simulink model "MMC_phase_centralized_HAAS_20260927"  (R2024b)
settings: Solver=FixedStepDiscrete  StartTime=t_init_sim  StopTime=sim_time  FixedStep=Ts  RelTol=1e-3
values from neighbouring files (symbols this model uses):
  a = 1    [script_MMC_phase_hackathon_NLM_centralized_HAAS_20260927.m]
  C1low1_active = 1    [script_MMC_phase_hackathon_NLM_centralized_HAAS_20260927.m]
  C2low1_active = 1    [script_MMC_phase_hackathon_NLM_centralized_HAAS_20260927.m]
  C_bus = 4400e-6    (= 0.0044)    [script_MMC_phase_hackathon_NLM_centralized_HAAS_20260927.m]
  C_M_extra = C_m-twist_high_side_C    [script_MMC_phase_hackathon_NLM_centralized_HAAS_20260927.m]
  duty_cycle = 1.0    (= 1)    [script_MMC_phase_hackathon_NLM_centralized_HAAS_20260927.m]
  f0 = 50    [script_MMC_phase_hackathon_NLM_centralized_HAAS_20260927.m]
  feeder_current_lower_rate_limit = -10    [script_MMC_phase_hackathon_NLM_centralized_HAAS_20260927.m]    (also in twist_parameters.m = -500)
  feeder_current_tab = [0.328 0.217 0.162 0.132 0.109 0.094 0.083 0.075 0.068 0.062 0.058 0.054 ... (42 elements, 14x3)]    [feeder_current.mat]
  feeder_current_upper_rate_limit = 0.386/(20e-3)    (= 19.3)    [twist_parameters.m]
  is6VExternallySupplied = true    [script_MMC_phase_hackathon_NLM_centralized_HAAS_20260927.m]
  isFeederJumperOpen = true    [script_MMC_phase_hackathon_NLM_centralized_HAAS_20260927.m]
  L_arm = 30e-3    (= 0.03)    [script_MMC_phase_hackathon_NLM_centralized_HAAS_20260927.m]
  m = 1    [script_MMC_phase_hackathon_NLM_centralized_HAAS_20260927.m]
  N = 5    [script_MMC_phase_hackathon_NLM_centralized_HAAS_20260927.m]
  power_losses = false    [script_MMC_phase_hackathon_NLM_centralized_HAAS_20260927.m]
  R = 15    [script_MMC_phase_hackathon_NLM_centralized_HAAS_20260927.m]
  R_arm = 0.2    [script_MMC_phase_hackathon_NLM_centralized_HAAS_20260927.m]
  source_V = 0    [script_MMC_phase_hackathon_NLM_centralized_HAAS_20260927.m]
  Tcom_sample = round(Tcom / Ts)    [script_MMC_phase_hackathon_NLM_centralized_HAAS_20260927.m]
  time_charge = 0.1    [script_MMC_phase_hackathon_NLM_centralized_HAAS_20260927.m]
  time_decharge = 1.5    [script_MMC_phase_hackathon_NLM_centralized_HAAS_20260927.m]
  Ts = 1e-6    (= 1e-06)    [script_MMC_phase_hackathon_NLM_centralized_HAAS_20260927.m]
  twist_data_acquisition_delay = 50e-9    (= 5e-08)    [script_MMC_phase_hackathon_NLM_centralized_HAAS_20260927.m]    (also in twist_parameters.m)
  twist_data_sampling_period = 1/twist_freq_data_sampling    (= 5e-05)    [script_MMC_phase_hackathon_NLM_centralized_HAAS_20260927.m]    (also in twist_parameters.m)
  twist_dead_time = 200e-9    (= 2e-07)    [twist_parameters.m]
  twist_freq_switching = 200e3    (= 200000)    [twist_parameters.m]
  twist_high_side_adc_R = 1/(1/2e6 + 1/2e6 + 1/(330e3+5.6e3))    (= 251272.836178)    [twist_parameters.m]
  twist_high_side_C = 33e-6*4 + 4.7e-6*12    (= 0.0001884)    [twist_parameters.m]
  twist_high_side_feeder_R = 47e3+4.7e3    (= 51700)    [twist_parameters.m]
  twist_high_side_rC = 0.1    [twist_parameters.m]
  twist_low_side_adc_R = 150e3+470    (= 150470)    [twist_parameters.m]
  twist_low_side_C_ceramic = 3*4.7e-6    (= 1.41e-05)    [twist_parameters.m]
  twist_low_side_C_electrolytic = 47e-6    (= 4.7e-05)    [twist_parameters.m]
  twist_low_side_L = 33e-6    (= 3.3e-05)    [twist_parameters.m]
  twist_low_side_rC = 700e-3    (= 0.7)    [twist_parameters.m]
  twist_low_side_rL = 20e-3    (= 0.02)    [twist_parameters.m]
  twist_R_VCC = (tau_VCC/twist_high_side_C  - twist_high_side_rC)/(1-(tau_VCC/twist_high_side_C - twist_high_side_rC)/R_parallel)    (= 1110.74997822)    [twist_parameters.m]
  VDC = 48    [script_MMC_phase_hackathon_NLM_centralized_HAAS_20260927.m]
undefined symbols (not defined in the file or in its folder): C_SM, feeder_current, gcbh, sps_rtmsupport, twist_low_side_lC
libraries: spsSeriesRLCBranchLib x135, spsTriangleGeneratorLib x60, spsMosfetLib x60, spsCurrentMeasurementLib x43, spsVoltageMeasurementLib x35, spsControlledCurrentSourceLib x30, spsDiodeLib x22, spsIdealSwitchLib x20, spsControlledVoltageSourceLib x1, spsGroundLib x1, spspowerguiLib x1
(part 10 of 22)

== system MMC_phase_centralized_HAAS_20260927/ /Subsystem/Subsystem/Hardware M2/Measurement block/i2Low acquisition ==
  In1 : Inport
  In2 : Inport  Port=2
  If : If  IfExpression=u1 > 0.99  ShowElse=off
  If Action Subsystem : Subsystem  TreatAsAtomicUnit=on
  Scope : Scope  NumInputPorts=3
  i2Meas : Outport
  wires:
  If Action Subsystem/1(Out1) -> Scope/1, i2Meas/1  "Data_Carry"
  In1/1 -> Scope/2, If Action Subsystem/1(In1)  "Data"
  If/1 -> If Action Subsystem/Action
  In2/1 -> If/1, Scope/3  "Carry"

== system MMC_phase_centralized_HAAS_20260927/ /Subsystem/Subsystem/Hardware M2/Measurement block/iHigh acquisition ==
  In1 : Inport
  In2 : Inport  Port=2
  If : If  IfExpression=u1 > 0.99  ShowElse=off
  If Action Subsystem : Subsystem  TreatAsAtomicUnit=on
  Scope : Scope  NumInputPorts=3
  iHMeas : Outport
  wires:
  If Action Subsystem/1(Out1) -> Scope/1, iHMeas/1  "Data_Carry"
  In1/1 -> Scope/2, If Action Subsystem/1(In1)  "Data"
  If/1 -> If Action Subsystem/Action
  In2/1 -> If/1, Scope/3  "Carry"

== system MMC_phase_centralized_HAAS_20260927/ /Subsystem/Subsystem/Hardware M2/Measurement block/v1Low acquisition ==
  In1 : Inport
  In2 : Inport  Port=2
  If : If  IfExpression=u1 > 0.99  ShowElse=off
  If Action Subsystem : Subsystem  TreatAsAtomicUnit=on
  Scope : Scope  NumInputPorts=3
  v1Meas : Outport
  wires:
  If Action Subsystem/1(Out1) -> Scope/1, v1Meas/1  "Data_Carry"
  In1/1 -> Scope/2, If Action Subsystem/1(In1)  "Data"
  If/1 -> If Action Subsystem/Action
  In2/1 -> If/1, Scope/3  "Carry"

== system MMC_phase_centralized_HAAS_20260927/ /Subsystem/Subsystem/Hardware M2/Measurement block/v2Low acquisition ==
  In1 : Inport
  In2 : Inport  Port=2
  If : If  IfExpression=u1 > 0.99  ShowElse=off
  If Action Subsystem : Subsystem  TreatAsAtomicUnit=on
  Scope : Scope  NumInputPorts=3
  v2Meas : Outport
  wires:
  If Action Subsystem/1(Out1) -> Scope/1, v2Meas/1  "Data_Carry"
  In1/1 -> Scope/2, If Action Subsystem/1(In1)  "Data"
  If/1 -> If Action Subsystem/Action
  In2/1 -> If/1, Scope/3  "Carry"

== system MMC_phase_centralized_HAAS_20260927/ /Subsystem/Subsystem/Hardware M2/Measurement block/vHigh acquisition ==
  In1 : Inport
  In2 : Inport  Port=2
  If : If  IfExpression=u1 > 0.99  ShowElse=off
  If Action Subsystem : Subsystem  TreatAsAtomicUnit=on
  Scope : Scope  NumInputPorts=3
  vHMeas : Outport
  wires:
  If Action Subsystem/1(Out1) -> Scope/1, vHMeas/1  "Data_Carry"
  In1/1 -> Scope/2, If Action Subsystem/1(In1)  "Data"
  If/1 -> If Action Subsystem/Action
  In2/1 -> If/1, Scope/3  "Carry"

== system MMC_phase_centralized_HAAS_20260927/ /Subsystem/Subsystem/Hardware M3/HRTimA_1/PWM Generator (2-Level) ==
  Uref : Inport  PortDimensions=sps.UrefInport_PortDimensions  SampleTime=Ts
  Bus Creator : BusCreator  Inputs=2
  Constant10 : Constant  Value=MinMax
  Cr_MinMax : Subsystem
  Data Type Conversion : DataTypeConversion  OutDataTypeStr=double  SaturateOnIntegerOverflow=off  RndMeth=Floor
  Logical Operator4 : Logic  Operator=NOT
  Modulator type : Subsystem  BlockChoice=One_Three_PhaseBridge  Variant=on  VariantControlMode=label  LabelModeActiveChoice=OneThreePhaseBridge
  Mux3 : Mux  Inputs=2
  Reference signal : Subsystem  BlockChoice=InternalUref  Variant=on  VariantControlMode=label  LabelModeActiveChoice=External
  Sampling : Subsystem  BlockChoice=Unsync_NaturalSampling  Variant=on  VariantControlMode=label  LabelModeActiveChoice=UnsyncSymmetrical
  Selector_Pout : Selector  InputPortWidth=sps.SelectorPout_PortSize  IndexOptions=Index vector (dialog)  Indices=sps.SelectorPout_Index  OutputSizes=1
  m : Terminator
  wt : Ground
  P : Outport  SampleTime=Ts  VectorParamsAs1DForOutWhenUnconnected=off
  Carry : Outport  Port=2  SampleTime=Ts  VectorParamsAs1DForOutWhenUnconnected=off
  wires:
  wt/1 -> Sampling/1(wt)
  Reference signal/1(Uref_In) -> Sampling/2(Uref)
  Modulator type/1(P) -> Logical Operator4/1, Mux3/1
  Constant10/1 -> Cr_MinMax/1(MinMax)
  Uref/1 -> Reference signal/1(Uref)
  Data Type Conversion/1 -> P/1
  Logical Operator4/1 -> Mux3/2
  Mux3/1 -> Selector_Pout/1
  Selector_Pout/1 -> Data Type Conversion/1
  Cr_MinMax/1(Cr*) -> Carry/1, Bus Creator/1, Modulator type/1(Cr)  "carrier"
  Sampling/1(Cr) -> Cr_MinMax/2(Cr)
  Sampling/2(Uref*) -> Bus Creator/2, Modulator type/2(Uref)  "Uref"
  Bus Creator/1 -> m/1

== system MMC_phase_centralized_HAAS_20260927/ /Subsystem/Subsystem/Hardware M3/HRTimA_2/PWM Generator (2-Level) ==
  Uref : Inport  PortDimensions=sps.UrefInport_PortDimensions  SampleTime=Ts
  Bus Creator : BusCreator  Inputs=2
  Constant10 : Constant  Value=MinMax
  Cr_MinMax : Subsystem
  Data Type Conversion : DataTypeConversion  OutDataTypeStr=double  SaturateOnIntegerOverflow=off  RndMeth=Floor
  Logical Operator4 : Logic  Operator=NOT
  Modulator type : Subsystem  BlockChoice=One_Three_PhaseBridge  Variant=on  VariantControlMode=label  LabelModeActiveChoice=OneThreePhaseBridge
  Mux3 : Mux  Inputs=2
  Reference signal : Subsystem  BlockChoice=InternalUref  Variant=on  VariantControlMode=label  LabelModeActiveChoice=External
  Sampling : Subsystem  BlockChoice=Unsync_NaturalSampling  Variant=on  VariantControlMode=label  LabelModeActiveChoice=UnsyncSymmetrical
  Selector_Pout : Selector  InputPortWidth=sps.SelectorPout_PortSize  IndexOptions=Index vector (dialog)  Indices=sps.SelectorPout_Index  OutputSizes=1
  m : Terminator
  wt : Ground
  P : Outport  SampleTime=Ts  VectorParamsAs1DForOutWhenUnconnected=off
  Carry : Outport  Port=2  SampleTime=Ts  VectorParamsAs1DForOutWhenUnconnected=off
  wires:
  wt/1 -> Sampling/1(wt)
  Reference signal/1(Uref_In) -> Sampling/2(Uref)
  Modulator type/1(P) -> Logical Operator4/1, Mux3/1
  Constant10/1 -> Cr_MinMax/1(MinMax)
  Uref/1 -> Reference signal/1(Uref)
  Data Type Conversion/1 -> P/1
  Logical Operator4/1 -> Mux3/2
  Mux3/1 -> Selector_Pout/1
  Selector_Pout/1 -> Data Type Conversion/1
  Cr_MinMax/1(Cr*) -> Carry/1, Bus Creator/1, Modulator type/1(Cr)  "carrier"
  Sampling/1(Cr) -> Cr_MinMax/2(Cr)
  Sampling/2(Uref*) -> Bus Creator/2, Modulator type/2(Uref)  "Uref"
  Bus Creator/1 -> m/1

== system MMC_phase_centralized_HAAS_20260927/ /Subsystem/Subsystem/Hardware M3/Measurement block/i1Low acquisition ==
  In1 : Inport
  In2 : Inport  Port=2
  If : If  IfExpression=u1 > 0.99  ShowElse=off
  If Action Subsystem : Subsystem  TreatAsAtomicUnit=on
  Scope : Scope  NumInputPorts=3
  i1Meas : Outport
  wires:
  If Action Subsystem/1(Out1) -> Scope/1, i1Meas/1  "Data_Carry"
  In1/1 -> Scope/2, If Action Subsystem/1(In1)  "Data"
  If/1 -> If Action Subsystem/Action
  In2/1 -> If/1, Scope/3  "Carry"

== system MMC_phase_centralized_HAAS_20260927/ /Subsystem/Subsystem/Hardware M3/Measurement block/i2Low acquisition ==
  In1 : Inport
  In2 : Inport  Port=2
  If : If  IfExpression=u1 > 0.99  ShowElse=off
  If Action Subsystem : Subsystem  TreatAsAtomicUnit=on
  Scope : Scope  NumInputPorts=3
  i2Meas : Outport
  wires:
  If Action Subsystem/1(Out1) -> Scope/1, i2Meas/1  "Data_Carry"
  In1/1 -> Scope/2, If Action Subsystem/1(In1)  "Data"
  If/1 -> If Action Subsystem/Action
  In2/1 -> If/1, Scope/3  "Carry"

== system MMC_phase_centralized_HAAS_20260927/ /Subsystem/Subsystem/Hardware M3/Measurement block/iHigh acquisition ==
  In1 : Inport
  In2 : Inport  Port=2
  If : If  IfExpression=u1 > 0.99  ShowElse=off
  If Action Subsystem : Subsystem  TreatAsAtomicUnit=on
  Scope : Scope  NumInputPorts=3
  iHMeas : Outport
  wires:
  If Action Subsystem/1(Out1) -> Scope/1, iHMeas/1  "Data_Carry"
  In1/1 -> Scope/2, If Action Subsystem/1(In1)  "Data"
  If/1 -> If Action Subsystem/Action
  In2/1 -> If/1, Scope/3  "Carry"

== system MMC_phase_centralized_HAAS_20260927/ /Subsystem/Subsystem/Hardware M3/Measurement block/v1Low acquisition ==
  In1 : Inport
  In2 : Inport  Port=2
  If : If  IfExpression=u1 > 0.99  ShowElse=off
  If Action Subsystem : Subsystem  TreatAsAtomicUnit=on
  Scope : Scope  NumInputPorts=3
  v1Meas : Outport
  wires:
  If Action Subsystem/1(Out1) -> Scope/1, v1Meas/1  "Data_Carry"
  In1/1 -> Scope/2, If Action Subsystem/1(In1)  "Data"
  If/1 -> If Action Subsystem/Action
  In2/1 -> If/1, Scope/3  "Carry"

== system MMC_phase_centralized_HAAS_20260927/ /Subsystem/Subsystem/Hardware M3/Measurement block/v2Low acquisition ==
  In1 : Inport
  In2 : Inport  Port=2
  If : If  IfExpression=u1 > 0.99  ShowElse=off
  If Action Subsystem : Subsystem  TreatAsAtomicUnit=on
  Scope : Scope  NumInputPorts=3
  v2Meas : Outport
  wires:
  If Action Subsystem/1(Out1) -> Scope/1, v2Meas/1  "Data_Carry"
  In1/1 -> Scope/2, If Action Subsystem/1(In1)  "Data"
  If/1 -> If Action Subsystem/Action
  In2/1 -> If/1, Scope/3  "Carry"

== system MMC_phase_centralized_HAAS_20260927/ /Subsystem/Subsystem/Hardware M3/Measurement block/vHigh acquisition ==
  In1 : Inport
  In2 : Inport  Port=2
  If : If  IfExpression=u1 > 0.99  ShowElse=off
  If Action Subsystem : Subsystem  TreatAsAtomicUnit=on
  Scope : Scope  NumInputPorts=3
  vHMeas : Outport
  wires:
  If Action Subsystem/1(Out1) -> Scope/1, vHMeas/1  "Data_Carry"
  In1/1 -> Scope/2, If Action Subsystem/1(In1)  "Data"
  If/1 -> If Action Subsystem/Action
  In2/1 -> If/1, Scope/3  "Carry"

== system MMC_phase_centralized_HAAS_20260927/ /Subsystem/Subsystem/Hardware M4/HRTimA_1/PWM Generator (2-Level) ==
  Uref : Inport  PortDimensions=sps.UrefInport_PortDimensions  SampleTime=Ts
  Bus Creator : BusCreator  Inputs=2
  Constant10 : Constant  Value=MinMax
  Cr_MinMax : Subsystem
  Data Type Conversion : DataTypeConversion  OutDataTypeStr=double  SaturateOnIntegerOverflow=off  RndMeth=Floor
  Logical Operator4 : Logic  Operator=NOT
  Modulator type : Subsystem  BlockChoice=One_Three_PhaseBridge  Variant=on  VariantControlMode=label  LabelModeActiveChoice=OneThreePhaseBridge
  Mux3 : Mux  Inputs=2
  Reference signal : Subsystem  BlockChoice=InternalUref  Variant=on  VariantControlMode=label  LabelModeActiveChoice=External
  Sampling : Subsystem  BlockChoice=Unsync_NaturalSampling  Variant=on  VariantControlMode=label  LabelModeActiveChoice=UnsyncSymmetrical
  Selector_Pout : Selector  InputPortWidth=sps.SelectorPout_PortSize  IndexOptions=Index vector (dialog)  Indices=sps.SelectorPout_Index  OutputSizes=1
  m : Terminator
  wt : Ground
  P : Outport  SampleTime=Ts  VectorParamsAs1DForOutWhenUnconnected=off
  Carry : Outport  Port=2  SampleTime=Ts  VectorParamsAs1DForOutWhenUnconnected=off
  wires:
  wt/1 -> Sampling/1(wt)
  Reference signal/1(Uref_In) -> Sampling/2(Uref)
  Modulator type/1(P) -> Logical Operator4/1, Mux3/1
  Constant10/1 -> Cr_MinMax/1(MinMax)
  Uref/1 -> Reference signal/1(Uref)
  Data Type Conversion/1 -> P/1
  Logical Operator4/1 -> Mux3/2
  Mux3/1 -> Selector_Pout/1
  Selector_Pout/1 -> Data Type Conversion/1
  Cr_MinMax/1(Cr*) -> Carry/1, Bus Creator/1, Modulator type/1(Cr)  "carrier"
  Sampling/1(Cr) -> Cr_MinMax/2(Cr)
  Sampling/2(Uref*) -> Bus Creator/2, Modulator type/2(Uref)  "Uref"
  Bus Creator/1 -> m/1

== system MMC_phase_centralized_HAAS_20260927/ /Subsystem/Subsystem/Hardware M4/HRTimA_2/PWM Generator (2-Level) ==
  Uref : Inport  PortDimensions=sps.UrefInport_PortDimensions  SampleTime=Ts
  Bus Creator : BusCreator  Inputs=2
  Constant10 : Constant  Value=MinMax
  Cr_MinMax : Subsystem
  Data Type Conversion : DataTypeConversion  OutDataTypeStr=double  SaturateOnIntegerOverflow=off  RndMeth=Floor
  Logical Operator4 : Logic  Operator=NOT
  Modulator type : Subsystem  BlockChoice=One_Three_PhaseBridge  Variant=on  VariantControlMode=label  LabelModeActiveChoice=OneThreePhaseBridge
  Mux3 : Mux  Inputs=2
  Reference signal : Subsystem  BlockChoice=InternalUref  Variant=on  VariantControlMode=label  LabelModeActiveChoice=External
  Sampling : Subsystem  BlockChoice=Unsync_NaturalSampling  Variant=on  VariantControlMode=label  LabelModeActiveChoice=UnsyncSymmetrical
  Selector_Pout : Selector  InputPortWidth=sps.SelectorPout_PortSize  IndexOptions=Index vector (dialog)  Indices=sps.SelectorPout_Index  OutputSizes=1
  m : Terminator
  wt : Ground
  P : Outport  SampleTime=Ts  VectorParamsAs1DForOutWhenUnconnected=off
  Carry : Outport  Port=2  SampleTime=Ts  VectorParamsAs1DForOutWhenUnconnected=off
  wires:
  wt/1 -> Sampling/1(wt)
  Reference signal/1(Uref_In) -> Sampling/2(Uref)
  Modulator type/1(P) -> Logical Operator4/1, Mux3/1
  Constant10/1 -> Cr_MinMax/1(MinMax)
  Uref/1 -> Reference signal/1(Uref)
  Data Type Conversion/1 -> P/1
  Logical Operator4/1 -> Mux3/2
  Mux3/1 -> Selector_Pout/1
  Selector_Pout/1 -> Data Type Conversion/1
  Cr_MinMax/1(Cr*) -> Carry/1, Bus Creator/1, Modulator type/1(Cr)  "carrier"
  Sampling/1(Cr) -> Cr_MinMax/2(Cr)
  Sampling/2(Uref*) -> Bus Creator/2, Modulator type/2(Uref)  "Uref"
  Bus Creator/1 -> m/1

== system MMC_phase_centralized_HAAS_20260927/ /Subsystem/Subsystem/Hardware M4/Measurement block/i1Low acquisition ==
  In1 : Inport
  In2 : Inport  Port=2
  If : If  IfExpression=u1 > 0.99  ShowElse=off
  If Action Subsystem : Subsystem  TreatAsAtomicUnit=on
  Scope : Scope  NumInputPorts=3
  i1Meas : Outport
  wires:
  If Action Subsystem/1(Out1) -> Scope/1, i1Meas/1  "Data_Carry"
  In1/1 -> Scope/2, If Action Subsystem/1(In1)  "Data"
  If/1 -> If Action Subsystem/Action
  In2/1 -> If/1, Scope/3  "Carry"

== system MMC_phase_centralized_HAAS_20260927/ /Subsystem/Subsystem/Hardware M4/Measurement block/i2Low acquisition ==
  In1 : Inport
  In2 : Inport  Port=2
  If : If  IfExpression=u1 > 0.99  ShowElse=off
  If Action Subsystem : Subsystem  TreatAsAtomicUnit=on
  Scope : Scope  NumInputPorts=3
  i2Meas : Outport
  wires:
  If Action Subsystem/1(Out1) -> Scope/1, i2Meas/1  "Data_Carry"
  In1/1 -> Scope/2, If Action Subsystem/1(In1)  "Data"
  If/1 -> If Action Subsystem/Action
  In2/1 -> If/1, Scope/3  "Carry"

== system MMC_phase_centralized_HAAS_20260927/ /Subsystem/Subsystem/Hardware M4/Measurement block/iHigh acquisition ==
  In1 : Inport
  In2 : Inport  Port=2
  If : If  IfExpression=u1 > 0.99  ShowElse=off
  If Action Subsystem : Subsystem  TreatAsAtomicUnit=on
  Scope : Scope  NumInputPorts=3
  iHMeas : Outport
  wires:
  If Action Subsystem/1(Out1) -> Scope/1, iHMeas/1  "Data_Carry"
  In1/1 -> Scope/2, If Action Subsystem/1(In1)  "Data"
  If/1 -> If Action Subsystem/Action
  In2/1 -> If/1, Scope/3  "Carry"

== system MMC_phase_centralized_HAAS_20260927/ /Subsystem/Subsystem/Hardware M4/Measurement block/v1Low acquisition ==
  In1 : Inport
  In2 : Inport  Port=2
  If : If  IfExpression=u1 > 0.99  ShowElse=off
  If Action Subsystem : Subsystem  TreatAsAtomicUnit=on
  Scope : Scope  NumInputPorts=3
  v1Meas : Outport
  wires:
  If Action Subsystem/1(Out1) -> Scope/1, v1Meas/1  "Data_Carry"
  In1/1 -> Scope/2, If Action Subsystem/1(In1)  "Data"
  If/1 -> If Action Subsystem/Action
  In2/1 -> If/1, Scope/3  "Carry"

== system MMC_phase_centralized_HAAS_20260927/ /Subsystem/Subsystem/Hardware M4/Measurement block/v2Low acquisition ==
  In1 : Inport
  In2 : Inport  Port=2
  If : If  IfExpression=u1 > 0.99  ShowElse=off
  If Action Subsystem : Subsystem  TreatAsAtomicUnit=on
  Scope : Scope  NumInputPorts=3
  v2Meas : Outport
  wires:
  If Action Subsystem/1(Out1) -> Scope/1, v2Meas/1  "Data_Carry"
  In1/1 -> Scope/2, If Action Subsystem/1(In1)  "Data"
  If/1 -> If Action Subsystem/Action
  In2/1 -> If/1, Scope/3  "Carry"

== system MMC_phase_centralized_HAAS_20260927/ /Subsystem/Subsystem/Hardware M4/Measurement block/vHigh acquisition ==
  In1 : Inport
  In2 : Inport  Port=2
  If : If  IfExpression=u1 > 0.99  ShowElse=off
  If Action Subsystem : Subsystem  TreatAsAtomicUnit=on
  Scope : Scope  NumInputPorts=3
  vHMeas : Outport
  wires:
  If Action Subsystem/1(Out1) -> Scope/1, vHMeas/1  "Data_Carry"
  In1/1 -> Scope/2, If Action Subsystem/1(In1)  "Data"
  If/1 -> If Action Subsystem/Action
  In2/1 -> If/1, Scope/3  "Carry"

== system MMC_phase_centralized_HAAS_20260927/ /Subsystem/Subsystem/Hardware M5/HRTimA_1/PWM Generator (2-Level) ==
  Uref : Inport  PortDimensions=sps.UrefInport_PortDimensions  SampleTime=Ts
  Bus Creator : BusCreator  Inputs=2
  Constant10 : Constant  Value=MinMax
  Cr_MinMax : Subsystem
  Data Type Conversion : DataTypeConversion  OutDataTypeStr=double  SaturateOnIntegerOverflow=off  RndMeth=Floor
  Logical Operator4 : Logic  Operator=NOT
  Modulator type : Subsystem  BlockChoice=One_Three_PhaseBridge  Variant=on  VariantControlMode=label  LabelModeActiveChoice=OneThreePhaseBridge
  Mux3 : Mux  Inputs=2
  Reference signal : Subsystem  BlockChoice=InternalUref  Variant=on  VariantControlMode=label  LabelModeActiveChoice=External
  Sampling : Subsystem  BlockChoice=Unsync_NaturalSampling  Variant=on  VariantControlMode=label  LabelModeActiveChoice=UnsyncSymmetrical
  Selector_Pout : Selector  InputPortWidth=sps.SelectorPout_PortSize  IndexOptions=Index vector (dialog)  Indices=sps.SelectorPout_Index  OutputSizes=1
  m : Terminator
  wt : Ground
  P : Outport  SampleTime=Ts  VectorParamsAs1DForOutWhenUnconnected=off
  Carry : Outport  Port=2  SampleTime=Ts  VectorParamsAs1DForOutWhenUnconnected=off
  wires:
  wt/1 -> Sampling/1(wt)
  Reference signal/1(Uref_In) -> Sampling/2(Uref)
  Modulator type/1(P) -> Logical Operator4/1, Mux3/1
  Constant10/1 -> Cr_MinMax/1(MinMax)
  Uref/1 -> Reference signal/1(Uref)
  Data Type Conversion/1 -> P/1
  Logical Operator4/1 -> Mux3/2
  Mux3/1 -> Selector_Pout/1
  Selector_Pout/1 -> Data Type Conversion/1
  Cr_MinMax/1(Cr*) -> Carry/1, Bus Creator/1, Modulator type/1(Cr)  "carrier"
  Sampling/1(Cr) -> Cr_MinMax/2(Cr)
  Sampling/2(Uref*) -> Bus Creator/2, Modulator type/2(Uref)  "Uref"
  Bus Creator/1 -> m/1

== system MMC_phase_centralized_HAAS_20260927/ /Subsystem/Subsystem/Hardware M5/HRTimA_2/PWM Generator (2-Level) ==
  Uref : Inport  PortDimensions=sps.UrefInport_PortDimensions  SampleTime=Ts
  Bus Creator : BusCreator  Inputs=2
  Constant10 : Constant  Value=MinMax
  Cr_MinMax : Subsystem
  Data Type Conversion : DataTypeConversion  OutDataTypeStr=double  SaturateOnIntegerOverflow=off  RndMeth=Floor
  Logical Operator4 : Logic  Operator=NOT
  Modulator type : Subsystem  BlockChoice=One_Three_PhaseBridge  Variant=on  VariantControlMode=label  LabelModeActiveChoice=OneThreePhaseBridge
  Mux3 : Mux  Inputs=2
  Reference signal : Subsystem  BlockChoice=InternalUref  Variant=on  VariantControlMode=label  LabelModeActiveChoice=External
  Sampling : Subsystem  BlockChoice=Unsync_NaturalSampling  Variant=on  VariantControlMode=label  LabelModeActiveChoice=UnsyncSymmetrical
  Selector_Pout : Selector  InputPortWidth=sps.SelectorPout_PortSize  IndexOptions=Index vector (dialog)  Indices=sps.SelectorPout_Index  OutputSizes=1
  m : Terminator
  wt : Ground
  P : Outport  SampleTime=Ts  VectorParamsAs1DForOutWhenUnconnected=off
  Carry : Outport  Port=2  SampleTime=Ts  VectorParamsAs1DForOutWhenUnconnected=off
  wires:
  wt/1 -> Sampling/1(wt)
  Reference signal/1(Uref_In) -> Sampling/2(Uref)
  Modulator type/1(P) -> Logical Operator4/1, Mux3/1
  Constant10/1 -> Cr_MinMax/1(MinMax)
  Uref/1 -> Reference signal/1(Uref)
  Data Type Conversion/1 -> P/1
  Logical Operator4/1 -> Mux3/2
  Mux3/1 -> Selector_Pout/1
  Selector_Pout/1 -> Data Type Conversion/1
  Cr_MinMax/1(Cr*) -> Carry/1, Bus Creator/1, Modulator type/1(Cr)  "carrier"
  Sampling/1(Cr) -> Cr_MinMax/2(Cr)
  Sampling/2(Uref*) -> Bus Creator/2, Modulator type/2(Uref)  "Uref"
  Bus Creator/1 -> m/1

== system MMC_phase_centralized_HAAS_20260927/ /Subsystem/Subsystem/Hardware M5/Measurement block/i1Low acquisition ==
  In1 : Inport
  In2 : Inport  Port=2
  If : If  IfExpression=u1 > 0.99  ShowElse=off
  If Action Subsystem : Subsystem  TreatAsAtomicUnit=on
  Scope : Scope  NumInputPorts=3
  i1Meas : Outport
  wires:
  If Action Subsystem/1(Out1) -> Scope/1, i1Meas/1  "Data_Carry"
  In1/1 -> Scope/2, If Action Subsystem/1(In1)  "Data"
  If/1 -> If Action Subsystem/Action
  In2/1 -> If/1, Scope/3  "Carry"

== system MMC_phase_centralized_HAAS_20260927/ /Subsystem/Subsystem/Hardware M5/Measurement block/i2Low acquisition ==
  In1 : Inport
  In2 : Inport  Port=2
  If : If  IfExpression=u1 > 0.99  ShowElse=off
  If Action Subsystem : Subsystem  TreatAsAtomicUnit=on
  Scope : Scope  NumInputPorts=3
  i2Meas : Outport
  wires:
  If Action Subsystem/1(Out1) -> Scope/1, i2Meas/1  "Data_Carry"
  In1/1 -> Scope/2, If Action Subsystem/1(In1)  "Data"
  If/1 -> If Action Subsystem/Action
  In2/1 -> If/1, Scope/3  "Carry"

== system MMC_phase_centralized_HAAS_20260927/ /Subsystem/Subsystem/Hardware M5/Measurement block/iHigh acquisition ==
  In1 : Inport
  In2 : Inport  Port=2
  If : If  IfExpression=u1 > 0.99  ShowElse=off
  If Action Subsystem : Subsystem  TreatAsAtomicUnit=on
  Scope : Scope  NumInputPorts=3
  iHMeas : Outport
  wires:
  If Action Subsystem/1(Out1) -> Scope/1, iHMeas/1  "Data_Carry"
  In1/1 -> Scope/2, If Action Subsystem/1(In1)  "Data"
  If/1 -> If Action Subsystem/Action
  In2/1 -> If/1, Scope/3  "Carry"

== system MMC_phase_centralized_HAAS_20260927/ /Subsystem/Subsystem/Hardware M5/Measurement block/v1Low acquisition ==
  In1 : Inport
  In2 : Inport  Port=2
  If : If  IfExpression=u1 > 0.99  ShowElse=off
  If Action Subsystem : Subsystem  TreatAsAtomicUnit=on
  Scope : Scope  NumInputPorts=3
  v1Meas : Outport
  wires:
  If Action Subsystem/1(Out1) -> Scope/1, v1Meas/1  "Data_Carry"
  In1/1 -> Scope/2, If Action Subsystem/1(In1)  "Data"
  If/1 -> If Action Subsystem/Action
  In2/1 -> If/1, Scope/3  "Carry"

== system MMC_phase_centralized_HAAS_20260927/ /Subsystem/Subsystem/Hardware M5/Measurement block/v2Low acquisition ==
  In1 : Inport
  In2 : Inport  Port=2
  If : If  IfExpression=u1 > 0.99  ShowElse=off
  If Action Subsystem : Subsystem  TreatAsAtomicUnit=on
  Scope : Scope  NumInputPorts=3
  v2Meas : Outport
  wires:
  If Action Subsystem/1(Out1) -> Scope/1, v2Meas/1  "Data_Carry"
  In1/1 -> Scope/2, If Action Subsystem/1(In1)  "Data"
  If/1 -> If Action Subsystem/Action
  In2/1 -> If/1, Scope/3  "Carry"

== system MMC_phase_centralized_HAAS_20260927/ /Subsystem/Subsystem/Hardware M5/Measurement block/vHigh acquisition ==
  In1 : Inport
  In2 : Inport  Port=2
  If : If  IfExpression=u1 > 0.99  ShowElse=off
  If Action Subsystem : Subsystem  TreatAsAtomicUnit=on
  Scope : Scope  NumInputPorts=3
  vHMeas : Outport
  wires:
  If Action Subsystem/1(Out1) -> Scope/1, vHMeas/1  "Data_Carry"
  In1/1 -> Scope/2, If Action Subsystem/1(In1)  "Data"
  If/1 -> If Action Subsystem/Action
  In2/1 -> If/1, Scope/3  "Carry"

== system MMC_phase_centralized_HAAS_20260927/ /Subsystem/Subsystem1/Hardware M1/HRTimA_1/PWM Generator (2-Level) ==
  Uref : Inport  PortDimensions=sps.UrefInport_PortDimensions  SampleTime=Ts
  Bus Creator : BusCreator  Inputs=2
  Constant10 : Constant  Value=MinMax
  Cr_MinMax : Subsystem
  Data Type Conversion : DataTypeConversion  OutDataTypeStr=double  SaturateOnIntegerOverflow=off  RndMeth=Floor
  Logical Operator4 : Logic  Operator=NOT
  Modulator type : Subsystem  BlockChoice=One_Three_PhaseBridge  Variant=on  VariantControlMode=label  LabelModeActiveChoice=OneThreePhaseBridge
  Mux3 : Mux  Inputs=2
  Reference signal : Subsystem  BlockChoice=InternalUref  Variant=on  VariantControlMode=label  LabelModeActiveChoice=External
  Sampling : Subsystem  BlockChoice=Unsync_NaturalSampling  Variant=on  VariantControlMode=label  LabelModeActiveChoice=UnsyncSymmetrical
  Selector_Pout : Selector  InputPortWidth=sps.SelectorPout_PortSize  IndexOptions=Index vector (dialog)  Indices=sps.SelectorPout_Index  OutputSizes=1
  m : Terminator
  wt : Ground
  P : Outport  SampleTime=Ts  VectorParamsAs1DForOutWhenUnconnected=off
  Carry : Outport  Port=2  SampleTime=Ts  VectorParamsAs1DForOutWhenUnconnected=off
  wires:
  wt/1 -> Sampling/1(wt)
  Reference signal/1(Uref_In) -> Sampling/2(Uref)
  Modulator type/1(P) -> Logical Operator4/1, Mux3/1
  Constant10/1 -> Cr_MinMax/1(MinMax)
  Uref/1 -> Reference signal/1(Uref)
  Data Type Conversion/1 -> P/1
  Logical Operator4/1 -> Mux3/2
  Mux3/1 -> Selector_Pout/1
  Selector_Pout/1 -> Data Type Conversion/1
  Cr_MinMax/1(Cr*) -> Carry/1, Bus Creator/1, Modulator type/1(Cr)  "carrier"
  Sampling/1(Cr) -> Cr_MinMax/2(Cr)
  Sampling/2(Uref*) -> Bus Creator/2, Modulator type/2(Uref)  "Uref"
  Bus Creator/1 -> m/1

== system MMC_phase_centralized_HAAS_20260927/ /Subsystem/Subsystem1/Hardware M1/HRTimA_2/PWM Generator (2-Level) ==
  Uref : Inport  PortDimensions=sps.UrefInport_PortDimensions  SampleTime=Ts
  Bus Creator : BusCreator  Inputs=2
  Constant10 : Constant  Value=MinMax
  Cr_MinMax : Subsystem
  Data Type Conversion : DataTypeConversion  OutDataTypeStr=double  SaturateOnIntegerOverflow=off  RndMeth=Floor
  Logical Operator4 : Logic  Operator=NOT
  Modulator type : Subsystem  BlockChoice=One_Three_PhaseBridge  Variant=on  VariantControlMode=label  LabelModeActiveChoice=OneThreePhaseBridge
  Mux3 : Mux  Inputs=2
  Reference signal : Subsystem  BlockChoice=InternalUref  Variant=on  VariantControlMode=label  LabelModeActiveChoice=External
  Sampling : Subsystem  BlockChoice=Unsync_NaturalSampling  Variant=on  VariantControlMode=label  LabelModeActiveChoice=UnsyncSymmetrical
  Selector_Pout : Selector  InputPortWidth=sps.SelectorPout_PortSize  IndexOptions=Index vector (dialog)  Indices=sps.SelectorPout_Index  OutputSizes=1
  m : Terminator
  wt : Ground
  P : Outport  SampleTime=Ts  VectorParamsAs1DForOutWhenUnconnected=off
  Carry : Outport  Port=2  SampleTime=Ts  VectorParamsAs1DForOutWhenUnconnected=off
  wires:
  wt/1 -> Sampling/1(wt)
  Reference signal/1(Uref_In) -> Sampling/2(Uref)
  Modulator type/1(P) -> Logical Operator4/1, Mux3/1
  Constant10/1 -> Cr_MinMax/1(MinMax)
  Uref/1 -> Reference signal/1(Uref)
  Data Type Conversion/1 -> P/1
  Logical Operator4/1 -> Mux3/2
  Mux3/1 -> Selector_Pout/1
  Selector_Pout/1 -> Data Type Conversion/1
  Cr_MinMax/1(Cr*) -> Carry/1, Bus Creator/1, Modulator type/1(Cr)  "carrier"
  Sampling/1(Cr) -> Cr_MinMax/2(Cr)
  Sampling/2(Uref*) -> Bus Creator/2, Modulator type/2(Uref)  "Uref"
  Bus Creator/1 -> m/1

== system MMC_phase_centralized_HAAS_20260927/ /Subsystem/Subsystem1/Hardware M1/Measurement block/i1Low acquisition ==
  In1 : Inport
  In2 : Inport  Port=2
  If : If  IfExpression=u1 > 0.99  ShowElse=off
  If Action Subsystem : Subsystem  TreatAsAtomicUnit=on
  Scope : Scope  NumInputPorts=3
  i1Meas : Outport
  wires:
  If Action Subsystem/1(Out1) -> Scope/1, i1Meas/1  "Data_Carry"
  In1/1 -> Scope/2, If Action Subsystem/1(In1)  "Data"
  If/1 -> If Action Subsystem/Action
  In2/1 -> If/1, Scope/3  "Carry"

== system MMC_phase_centralized_HAAS_20260927/ /Subsystem/Subsystem1/Hardware M1/Measurement block/i2Low acquisition ==
  In1 : Inport
  In2 : Inport  Port=2
  If : If  IfExpression=u1 > 0.99  ShowElse=off
  If Action Subsystem : Subsystem  TreatAsAtomicUnit=on
  Scope : Scope  NumInputPorts=3
  i2Meas : Outport
  wires:
  If Action Subsystem/1(Out1) -> Scope/1, i2Meas/1  "Data_Carry"
  In1/1 -> Scope/2, If Action Subsystem/1(In1)  "Data"
  If/1 -> If Action Subsystem/Action
  In2/1 -> If/1, Scope/3  "Carry"

== system MMC_phase_centralized_HAAS_20260927/ /Subsystem/Subsystem1/Hardware M1/Measurement block/iHigh acquisition ==
  In1 : Inport
  In2 : Inport  Port=2
  If : If  IfExpression=u1 > 0.99  ShowElse=off
  If Action Subsystem : Subsystem  TreatAsAtomicUnit=on
  Scope : Scope  NumInputPorts=3
  iHMeas : Outport
  wires:
  If Action Subsystem/1(Out1) -> Scope/1, iHMeas/1  "Data_Carry"
  In1/1 -> Scope/2, If Action Subsystem/1(In1)  "Data"
  If/1 -> If Action Subsystem/Action
  In2/1 -> If/1, Scope/3  "Carry"

== system MMC_phase_centralized_HAAS_20260927/ /Subsystem/Subsystem1/Hardware M1/Measurement block/v1Low acquisition ==
  In1 : Inport
  In2 : Inport  Port=2
  If : If  IfExpression=u1 > 0.99  ShowElse=off
  If Action Subsystem : Subsystem  TreatAsAtomicUnit=on
  Scope : Scope  NumInputPorts=3
  v1Meas : Outport
  wires:
  If Action Subsystem/1(Out1) -> Scope/1, v1Meas/1  "Data_Carry"
  In1/1 -> Scope/2, If Action Subsystem/1(In1)  "Data"
  If/1 -> If Action Subsystem/Action
  In2/1 -> If/1, Scope/3  "Carry"

== system MMC_phase_centralized_HAAS_20260927/ /Subsystem/Subsystem1/Hardware M1/Measurement block/v2Low acquisition ==
  In1 : Inport
  In2 : Inport  Port=2
  If : If  IfExpression=u1 > 0.99  ShowElse=off
  If Action Subsystem : Subsystem  TreatAsAtomicUnit=on
  Scope : Scope  NumInputPorts=3
  v2Meas : Outport
  wires:
  If Action Subsystem/1(Out1) -> Scope/1, v2Meas/1  "Data_Carry"
  In1/1 -> Scope/2, If Action Subsystem/1(In1)  "Data"
  If/1 -> If Action Subsystem/Action
  In2/1 -> If/1, Scope/3  "Carry"

== system MMC_phase_centralized_HAAS_20260927/ /Subsystem/Subsystem1/Hardware M1/Measurement block/vHigh acquisition ==
  In1 : Inport
  In2 : Inport  Port=2
  If : If  IfExpression=u1 > 0.99  ShowElse=off
  If Action Subsystem : Subsystem  TreatAsAtomicUnit=on
  Scope : Scope  NumInputPorts=3
  vHMeas : Outport
  wires:
  If Action Subsystem/1(Out1) -> Scope/1, vHMeas/1  "Data_Carry"
  In1/1 -> Scope/2, If Action Subsystem/1(In1)  "Data"
  If/1 -> If Action Subsystem/Action
  In2/1 -> If/1, Scope/3  "Carry"

== system MMC_phase_centralized_HAAS_20260927/ /Subsystem/Subsystem1/Hardware M2/HRTimA_1/PWM Generator (2-Level) ==
  Uref : Inport  PortDimensions=sps.UrefInport_PortDimensions  SampleTime=Ts
  Bus Creator : BusCreator  Inputs=2
  Constant10 : Constant  Value=MinMax
  Cr_MinMax : Subsystem
  Data Type Conversion : DataTypeConversion  OutDataTypeStr=double  SaturateOnIntegerOverflow=off  RndMeth=Floor
  Logical Operator4 : Logic  Operator=NOT
  Modulator type : Subsystem  BlockChoice=One_Three_PhaseBridge  Variant=on  VariantControlMode=label  LabelModeActiveChoice=OneThreePhaseBridge
  Mux3 : Mux  Inputs=2
  Reference signal : Subsystem  BlockChoice=InternalUref  Variant=on  VariantControlMode=label  LabelModeActiveChoice=External
  Sampling : Subsystem  BlockChoice=Unsync_NaturalSampling  Variant=on  VariantControlMode=label  LabelModeActiveChoice=UnsyncSymmetrical
  Selector_Pout : Selector  InputPortWidth=sps.SelectorPout_PortSize  IndexOptions=Index vector (dialog)  Indices=sps.SelectorPout_Index  OutputSizes=1
  m : Terminator
  wt : Ground
  P : Outport  SampleTime=Ts  VectorParamsAs1DForOutWhenUnconnected=off
  Carry : Outport  Port=2  SampleTime=Ts  VectorParamsAs1DForOutWhenUnconnected=off
  wires:
  wt/1 -> Sampling/1(wt)
  Reference signal/1(Uref_In) -> Sampling/2(Uref)
  Modulator type/1(P) -> Logical Operator4/1, Mux3/1
  Constant10/1 -> Cr_MinMax/1(MinMax)
  Uref/1 -> Reference signal/1(Uref)
  Data Type Conversion/1 -> P/1
  Logical Operator4/1 -> Mux3/2
  Mux3/1 -> Selector_Pout/1
  Selector_Pout/1 -> Data Type Conversion/1
  Cr_MinMax/1(Cr*) -> Carry/1, Bus Creator/1, Modulator type/1(Cr)  "carrier"
  Sampling/1(Cr) -> Cr_MinMax/2(Cr)
  Sampling/2(Uref*) -> Bus Creator/2, Modulator type/2(Uref)  "Uref"
  Bus Creator/1 -> m/1

== system MMC_phase_centralized_HAAS_20260927/ /Subsystem/Subsystem1/Hardware M2/HRTimA_2/PWM Generator (2-Level) ==
  Uref : Inport  PortDimensions=sps.UrefInport_PortDimensions  SampleTime=Ts
  Bus Creator : BusCreator  Inputs=2
  Constant10 : Constant  Value=MinMax
  Cr_MinMax : Subsystem
  Data Type Conversion : DataTypeConversion  OutDataTypeStr=double  SaturateOnIntegerOverflow=off  RndMeth=Floor
  Logical Operator4 : Logic  Operator=NOT
  Modulator type : Subsystem  BlockChoice=One_Three_PhaseBridge  Variant=on  VariantControlMode=label  LabelModeActiveChoice=OneThreePhaseBridge
  Mux3 : Mux  Inputs=2
  Reference signal : Subsystem  BlockChoice=InternalUref  Variant=on  VariantControlMode=label  LabelModeActiveChoice=External
  Sampling : Subsystem  BlockChoice=Unsync_NaturalSampling  Variant=on  VariantControlMode=label  LabelModeActiveChoice=UnsyncSymmetrical
  Selector_Pout : Selector  InputPortWidth=sps.SelectorPout_PortSize  IndexOptions=Index vector (dialog)  Indices=sps.SelectorPout_Index  OutputSizes=1
  m : Terminator
  wt : Ground
  P : Outport  SampleTime=Ts  VectorParamsAs1DForOutWhenUnconnected=off
  Carry : Outport  Port=2  SampleTime=Ts  VectorParamsAs1DForOutWhenUnconnected=off
  wires:
  wt/1 -> Sampling/1(wt)
  Reference signal/1(Uref_In) -> Sampling/2(Uref)
  Modulator type/1(P) -> Logical Operator4/1, Mux3/1
  Constant10/1 -> Cr_MinMax/1(MinMax)
  Uref/1 -> Reference signal/1(Uref)
  Data Type Conversion/1 -> P/1
  Logical Operator4/1 -> Mux3/2
  Mux3/1 -> Selector_Pout/1
  Selector_Pout/1 -> Data Type Conversion/1
  Cr_MinMax/1(Cr*) -> Carry/1, Bus Creator/1, Modulator type/1(Cr)  "carrier"
  Sampling/1(Cr) -> Cr_MinMax/2(Cr)
  Sampling/2(Uref*) -> Bus Creator/2, Modulator type/2(Uref)  "Uref"
  Bus Creator/1 -> m/1

== system MMC_phase_centralized_HAAS_20260927/ /Subsystem/Subsystem1/Hardware M2/Measurement block/i1Low acquisition ==
  In1 : Inport
  In2 : Inport  Port=2
  If : If  IfExpression=u1 > 0.99  ShowElse=off
  If Action Subsystem : Subsystem  TreatAsAtomicUnit=on
  Scope : Scope  NumInputPorts=3
  i1Meas : Outport
  wires:
  If Action Subsystem/1(Out1) -> Scope/1, i1Meas/1  "Data_Carry"
  In1/1 -> Scope/2, If Action Subsystem/1(In1)  "Data"
  If/1 -> If Action Subsystem/Action
  In2/1 -> If/1, Scope/3  "Carry"

== system MMC_phase_centralized_HAAS_20260927/ /Subsystem/Subsystem1/Hardware M2/Measurement block/i2Low acquisition ==
  In1 : Inport
  In2 : Inport  Port=2
  If : If  IfExpression=u1 > 0.99  ShowElse=off
  If Action Subsystem : Subsystem  TreatAsAtomicUnit=on
  Scope : Scope  NumInputPorts=3
  i2Meas : Outport
  wires:
  If Action Subsystem/1(Out1) -> Scope/1, i2Meas/1  "Data_Carry"
  In1/1 -> Scope/2, If Action Subsystem/1(In1)  "Data"
  If/1 -> If Action Subsystem/Action
  In2/1 -> If/1, Scope/3  "Carry"

== system MMC_phase_centralized_HAAS_20260927/ /Subsystem/Subsystem1/Hardware M2/Measurement block/iHigh acquisition ==
  In1 : Inport
  In2 : Inport  Port=2
  If : If  IfExpression=u1 > 0.99  ShowElse=off
  If Action Subsystem : Subsystem  TreatAsAtomicUnit=on
  Scope : Scope  NumInputPorts=3
  iHMeas : Outport
  wires:
  If Action Subsystem/1(Out1) -> Scope/1, iHMeas/1  "Data_Carry"
  In1/1 -> Scope/2, If Action Subsystem/1(In1)  "Data"
  If/1 -> If Action Subsystem/Action
  In2/1 -> If/1, Scope/3  "Carry"

== system MMC_phase_centralized_HAAS_20260927/ /Subsystem/Subsystem1/Hardware M2/Measurement block/v1Low acquisition ==
  In1 : Inport
  In2 : Inport  Port=2
  If : If  IfExpression=u1 > 0.99  ShowElse=off
  If Action Subsystem : Subsystem  TreatAsAtomicUnit=on
  Scope : Scope  NumInputPorts=3
  v1Meas : Outport
  wires:
  If Action Subsystem/1(Out1) -> Scope/1, v1Meas/1  "Data_Carry"
  In1/1 -> Scope/2, If Action Subsystem/1(In1)  "Data"
  If/1 -> If Action Subsystem/Action
  In2/1 -> If/1, Scope/3  "Carry"

== system MMC_phase_centralized_HAAS_20260927/ /Subsystem/Subsystem1/Hardware M2/Measurement block/v2Low acquisition ==
  In1 : Inport
  In2 : Inport  Port=2
  If : If  IfExpression=u1 > 0.99  ShowElse=off
  If Action Subsystem : Subsystem  TreatAsAtomicUnit=on
  Scope : Scope  NumInputPorts=3
  v2Meas : Outport
  wires:
  If Action Subsystem/1(Out1) -> Scope/1, v2Meas/1  "Data_Carry"
  In1/1 -> Scope/2, If Action Subsystem/1(In1)  "Data"
  If/1 -> If Action Subsystem/Action
  In2/1 -> If/1, Scope/3  "Carry"

== system MMC_phase_centralized_HAAS_20260927/ /Subsystem/Subsystem1/Hardware M2/Measurement block/vHigh acquisition ==
  In1 : Inport
  In2 : Inport  Port=2
  If : If  IfExpression=u1 > 0.99  ShowElse=off
  If Action Subsystem : Subsystem  TreatAsAtomicUnit=on
  Scope : Scope  NumInputPorts=3
  vHMeas : Outport
  wires:
  If Action Subsystem/1(Out1) -> Scope/1, vHMeas/1  "Data_Carry"
  In1/1 -> Scope/2, If Action Subsystem/1(In1)  "Data"
  If/1 -> If Action Subsystem/Action
  In2/1 -> If/1, Scope/3  "Carry"

== system MMC_phase_centralized_HAAS_20260927/ /Subsystem/Subsystem1/Hardware M3/HRTimA_1/PWM Generator (2-Level) ==
  Uref : Inport  PortDimensions=sps.UrefInport_PortDimensions  SampleTime=Ts
  Bus Creator : BusCreator  Inputs=2
  Constant10 : Constant  Value=MinMax
  Cr_MinMax : Subsystem
  Data Type Conversion : DataTypeConversion  OutDataTypeStr=double  SaturateOnIntegerOverflow=off  RndMeth=Floor
  Logical Operator4 : Logic  Operator=NOT
  Modulator type : Subsystem  BlockChoice=One_Three_PhaseBridge  Variant=on  VariantControlMode=label  LabelModeActiveChoice=OneThreePhaseBridge
  Mux3 : Mux  Inputs=2
  Reference signal : Subsystem  BlockChoice=InternalUref  Variant=on  VariantControlMode=label  LabelModeActiveChoice=External
  Sampling : Subsystem  BlockChoice=Unsync_NaturalSampling  Variant=on  VariantControlMode=label  LabelModeActiveChoice=UnsyncSymmetrical
  Selector_Pout : Selector  InputPortWidth=sps.SelectorPout_PortSize  IndexOptions=Index vector (dialog)  Indices=sps.SelectorPout_Index  OutputSizes=1
  m : Terminator
  wt : Ground
  P : Outport  SampleTime=Ts  VectorParamsAs1DForOutWhenUnconnected=off
  Carry : Outport  Port=2  SampleTime=Ts  VectorParamsAs1DForOutWhenUnconnected=off
  wires:
  wt/1 -> Sampling/1(wt)
  Reference signal/1(Uref_In) -> Sampling/2(Uref)
  Modulator type/1(P) -> Logical Operator4/1, Mux3/1
  Constant10/1 -> Cr_MinMax/1(MinMax)
  Uref/1 -> Reference signal/1(Uref)
  Data Type Conversion/1 -> P/1
  Logical Operator4/1 -> Mux3/2
  Mux3/1 -> Selector_Pout/1
  Selector_Pout/1 -> Data Type Conversion/1
  Cr_MinMax/1(Cr*) -> Carry/1, Bus Creator/1, Modulator type/1(Cr)  "carrier"
  Sampling/1(Cr) -> Cr_MinMax/2(Cr)
  Sampling/2(Uref*) -> Bus Creator/2, Modulator type/2(Uref)  "Uref"
  Bus Creator/1 -> m/1

== system MMC_phase_centralized_HAAS_20260927/ /Subsystem/Subsystem1/Hardware M3/HRTimA_2/PWM Generator (2-Level) ==
  Uref : Inport  PortDimensions=sps.UrefInport_PortDimensions  SampleTime=Ts
  Bus Creator : BusCreator  Inputs=2
  Constant10 : Constant  Value=MinMax
  Cr_MinMax : Subsystem
  Data Type Conversion : DataTypeConversion  OutDataTypeStr=double  SaturateOnIntegerOverflow=off  RndMeth=Floor
  Logical Operator4 : Logic  Operator=NOT
  Modulator type : Subsystem  BlockChoice=One_Three_PhaseBridge  Variant=on  VariantControlMode=label  LabelModeActiveChoice=OneThreePhaseBridge
  Mux3 : Mux  Inputs=2
  Reference signal : Subsystem  BlockChoice=InternalUref  Variant=on  VariantControlMode=label  LabelModeActiveChoice=External
  Sampling : Subsystem  BlockChoice=Unsync_NaturalSampling  Variant=on  VariantControlMode=label  LabelModeActiveChoice=UnsyncSymmetrical
  Selector_Pout : Selector  InputPortWidth=sps.SelectorPout_PortSize  IndexOptions=Index vector (dialog)  Indices=sps.SelectorPout_Index  OutputSizes=1
  m : Terminator
  wt : Ground
  P : Outport  SampleTime=Ts  VectorParamsAs1DForOutWhenUnconnected=off
  Carry : Outport  Port=2  SampleTime=Ts  VectorParamsAs1DForOutWhenUnconnected=off
  wires:
  wt/1 -> Sampling/1(wt)
  Reference signal/1(Uref_In) -> Sampling/2(Uref)
  Modulator type/1(P) -> Logical Operator4/1, Mux3/1
  Constant10/1 -> Cr_MinMax/1(MinMax)
  Uref/1 -> Reference signal/1(Uref)
  Data Type Conversion/1 -> P/1
  Logical Operator4/1 -> Mux3/2
  Mux3/1 -> Selector_Pout/1
  Selector_Pout/1 -> Data Type Conversion/1
  Cr_MinMax/1(Cr*) -> Carry/1, Bus Creator/1, Modulator type/1(Cr)  "carrier"
  Sampling/1(Cr) -> Cr_MinMax/2(Cr)
  Sampling/2(Uref*) -> Bus Creator/2, Modulator type/2(Uref)  "Uref"
  Bus Creator/1 -> m/1

== system MMC_phase_centralized_HAAS_20260927/ /Subsystem/Subsystem1/Hardware M3/Measurement block/i1Low acquisition ==
  In1 : Inport
  In2 : Inport  Port=2
  If : If  IfExpression=u1 > 0.99  ShowElse=off
  If Action Subsystem : Subsystem  TreatAsAtomicUnit=on
  Scope : Scope  NumInputPorts=3
  i1Meas : Outport
  wires:
  If Action Subsystem/1(Out1) -> Scope/1, i1Meas/1  "Data_Carry"
  In1/1 -> Scope/2, If Action Subsystem/1(In1)  "Data"
  If/1 -> If Action Subsystem/Action
  In2/1 -> If/1, Scope/3  "Carry"

== system MMC_phase_centralized_HAAS_20260927/ /Subsystem/Subsystem1/Hardware M3/Measurement block/i2Low acquisition ==
  In1 : Inport
  In2 : Inport  Port=2
  If : If  IfExpression=u1 > 0.99  ShowElse=off
  If Action Subsystem : Subsystem  TreatAsAtomicUnit=on
  Scope : Scope  NumInputPorts=3
  i2Meas : Outport
  wires:
  If Action Subsystem/1(Out1) -> Scope/1, i2Meas/1  "Data_Carry"
  In1/1 -> Scope/2, If Action Subsystem/1(In1)  "Data"
  If/1 -> If Action Subsystem/Action
  In2/1 -> If/1, Scope/3  "Carry"

== system MMC_phase_centralized_HAAS_20260927/ /Subsystem/Subsystem1/Hardware M3/Measurement block/iHigh acquisition ==
  In1 : Inport
  In2 : Inport  Port=2
  If : If  IfExpression=u1 > 0.99  ShowElse=off
  If Action Subsystem : Subsystem  TreatAsAtomicUnit=on
  Scope : Scope  NumInputPorts=3
  iHMeas : Outport
  wires:
  If Action Subsystem/1(Out1) -> Scope/1, iHMeas/1  "Data_Carry"
  In1/1 -> Scope/2, If Action Subsystem/1(In1)  "Data"
  If/1 -> If Action Subsystem/Action
  In2/1 -> If/1, Scope/3  "Carry"

== system MMC_phase_centralized_HAAS_20260927/ /Subsystem/Subsystem1/Hardware M3/Measurement block/v1Low acquisition ==
  In1 : Inport
  In2 : Inport  Port=2
  If : If  IfExpression=u1 > 0.99  ShowElse=off
  If Action Subsystem : Subsystem  TreatAsAtomicUnit=on
  Scope : Scope  NumInputPorts=3
  v1Meas : Outport
  wires:
  If Action Subsystem/1(Out1) -> Scope/1, v1Meas/1  "Data_Carry"
  In1/1 -> Scope/2, If Action Subsystem/1(In1)  "Data"
  If/1 -> If Action Subsystem/Action
  In2/1 -> If/1, Scope/3  "Carry"

== system MMC_phase_centralized_HAAS_20260927/ /Subsystem/Subsystem1/Hardware M3/Measurement block/v2Low acquisition ==
  In1 : Inport
  In2 : Inport  Port=2
  If : If  IfExpression=u1 > 0.99  ShowElse=off
  If Action Subsystem : Subsystem  TreatAsAtomicUnit=on
  Scope : Scope  NumInputPorts=3
  v2Meas : Outport
  wires:
  If Action Subsystem/1(Out1) -> Scope/1, v2Meas/1  "Data_Carry"
  In1/1 -> Scope/2, If Action Subsystem/1(In1)  "Data"
  If/1 -> If Action Subsystem/Action
  In2/1 -> If/1, Scope/3  "Carry"

== system MMC_phase_centralized_HAAS_20260927/ /Subsystem/Subsystem1/Hardware M3/Measurement block/vHigh acquisition ==
  In1 : Inport
  In2 : Inport  Port=2
  If : If  IfExpression=u1 > 0.99  ShowElse=off
  If Action Subsystem : Subsystem  TreatAsAtomicUnit=on
  Scope : Scope  NumInputPorts=3
  vHMeas : Outport
  wires:
  If Action Subsystem/1(Out1) -> Scope/1, vHMeas/1  "Data_Carry"
  In1/1 -> Scope/2, If Action Subsystem/1(In1)  "Data"
  If/1 -> If Action Subsystem/Action
  In2/1 -> If/1, Scope/3  "Carry"

== system MMC_phase_centralized_HAAS_20260927/ /Subsystem/Subsystem1/Hardware M4/HRTimA_1/PWM Generator (2-Level) ==
  Uref : Inport  PortDimensions=sps.UrefInport_PortDimensions  SampleTime=Ts
  Bus Creator : BusCreator  Inputs=2
  Constant10 : Constant  Value=MinMax
  Cr_MinMax : Subsystem
  Data Type Conversion : DataTypeConversion  OutDataTypeStr=double  SaturateOnIntegerOverflow=off  RndMeth=Floor
  Logical Operator4 : Logic  Operator=NOT
  Modulator type : Subsystem  BlockChoice=One_Three_PhaseBridge  Variant=on  VariantControlMode=label  LabelModeActiveChoice=OneThreePhaseBridge
  Mux3 : Mux  Inputs=2
  Reference signal : Subsystem  BlockChoice=InternalUref  Variant=on  VariantControlMode=label  LabelModeActiveChoice=External
  Sampling : Subsystem  BlockChoice=Unsync_NaturalSampling  Variant=on  VariantControlMode=label  LabelModeActiveChoice=UnsyncSymmetrical
  Selector_Pout : Selector  InputPortWidth=sps.SelectorPout_PortSize  IndexOptions=Index vector (dialog)  Indices=sps.SelectorPout_Index  OutputSizes=1
  m : Terminator
  wt : Ground
  P : Outport  SampleTime=Ts  VectorParamsAs1DForOutWhenUnconnected=off
  Carry : Outport  Port=2  SampleTime=Ts  VectorParamsAs1DForOutWhenUnconnected=off
  wires:
  wt/1 -> Sampling/1(wt)
  Reference signal/1(Uref_In) -> Sampling/2(Uref)
  Modulator type/1(P) -> Logical Operator4/1, Mux3/1
  Constant10/1 -> Cr_MinMax/1(MinMax)
  Uref/1 -> Reference signal/1(Uref)
  Data Type Conversion/1 -> P/1
  Logical Operator4/1 -> Mux3/2
  Mux3/1 -> Selector_Pout/1
  Selector_Pout/1 -> Data Type Conversion/1
  Cr_MinMax/1(Cr*) -> Carry/1, Bus Creator/1, Modulator type/1(Cr)  "carrier"
  Sampling/1(Cr) -> Cr_MinMax/2(Cr)
  Sampling/2(Uref*) -> Bus Creator/2, Modulator type/2(Uref)  "Uref"
  Bus Creator/1 -> m/1
